simulink model "four_quadrant_chopper"  (R2024b)
settings: Solver=FixedStepAuto  StartTime=0.0  StopTime=1  FixedStep=1e-06  MaxStep=1e-6  RelTol=1e-3
values from neighbouring files (symbols this model uses):
  fsw = 100000    [parameters.m]
  Is = 102    [parameters.m]
  J = Jl + Jr    (= 3.48e-05)    [parameters.m]
  kt = 0.0164    [parameters.m]
  kw = ks*30/pi    (= 5548.14131618)    [parameters.m]
  R = 0.12    [parameters.m]
  Ri = 0.1    [parameters.m]
  Rii = 1000    [parameters.m]
  Rp = 0.02    [parameters.m]
  Rpi = 50    [parameters.m]
  Rv = 0.15    [parameters.m]
  slt = 0.00002848    (= 2.848e-05)    [parameters.m]
  V = 15    [parameters.m]
  vn = 6370    [parameters.m]
libraries: nesl_utility x12, ee_lib x10, fl_lib x8, simulink x2
settings Model: Creator=Samuele  LastModifiedBy=tommymagelli
settings SolverCC: ZeroCrossAlgorithm=Adaptive
settings DebuggingCC: IgnoredZcDiagnostic=none
settings RTWCC: GPUComputeCapability=3.5

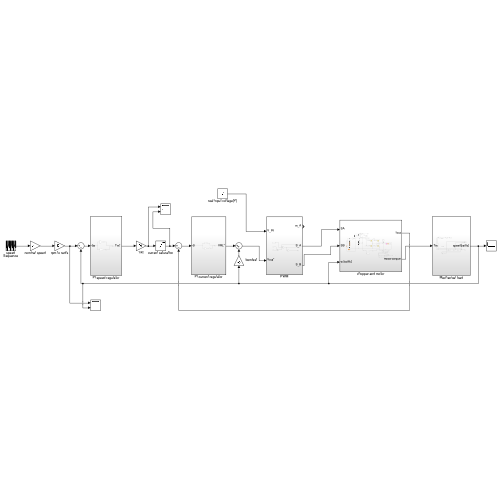
[thumbnail: Simulink's stored preview of the top-level diagram]
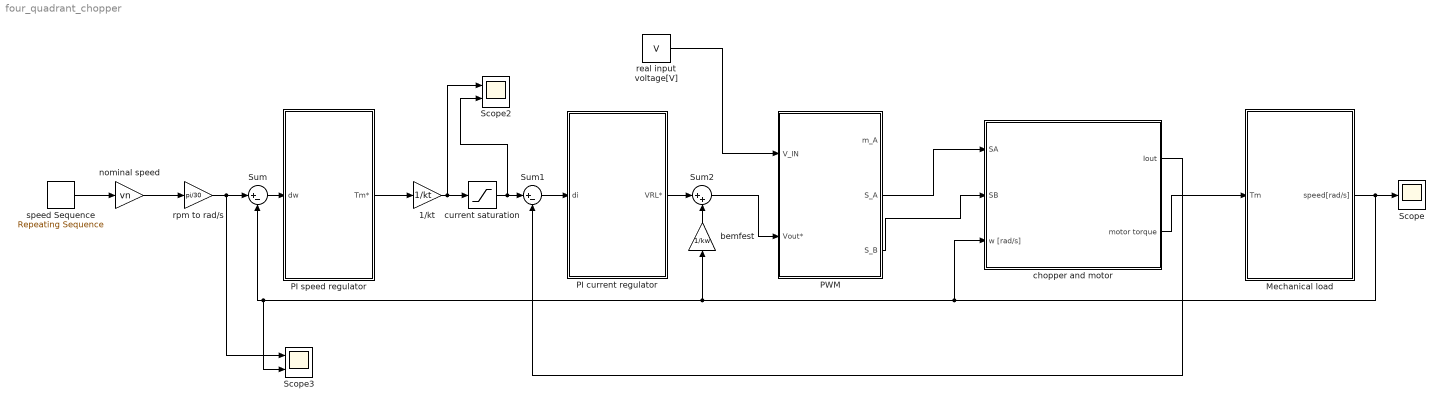
== system four_quadrant_chopper ==
  1/kt : Gain  Gain=1/kt
  Mechanical load : Subsystem
  PI current regulator : Subsystem
  PI speed regulator : Subsystem
  PWM : Subsystem
  Scope : Scope
  Scope2 : Scope  NumInputPorts=2
  Scope3 : Scope  NumInputPorts=2
  Sum : Sum  Inputs=|+-
  Sum1 : Sum  Inputs=|+-
  Sum2 : Sum  Inputs=|++
  bemfest : Gain  Gain=1/kw
  chopper and motor : Subsystem
  current saturation : Saturate  UpperLimit=Is  LowerLimit=-Is
  nominal speed : Gain  Gain=vn
  real input voltage[V] : Constant  Value=V
  rpm to rad/s : Gain  Gain=pi/30
  speed Sequence : simulink/Sources/Repeating Sequence  rep_seq_t=time  rep_seq_y=value
  wires:
  Sum1/1 -> PI current regulator/1(di)
  1/kt/1 -> Scope2/1, current saturation/1
  real input voltage[V]/1 -> PWM/1(V_IN)
  PI speed regulator/1(Tm*) -> 1/kt/1
  Sum2/1 -> PWM/2(Vout*)
  PI current regulator/1(VRL*) -> Sum2/1
  current saturation/1 -> Scope2/2, Sum1/1
  Sum/1 -> PI speed regulator/1(dw)
  rpm to rad/s/1 -> Scope3/1, Sum/1
  speed Sequence/1 -> nominal speed/1
  Mechanical load/1(speed[rad/s]) -> chopper and motor/3(w [rad/s]), Scope3/2, Sum/2, bemfest/1, Scope/1
  nominal speed/1 -> rpm to rad/s/1
  bemfest/1 -> Sum2/2
  chopper and motor/1(Iout) -> Sum1/2
  chopper and motor/2(motor torque) -> Mechanical load/1(Tm)
  PWM/2(S_A) -> chopper and motor/1(SA)
  PWM/3(S_B) -> chopper and motor/2(SB)

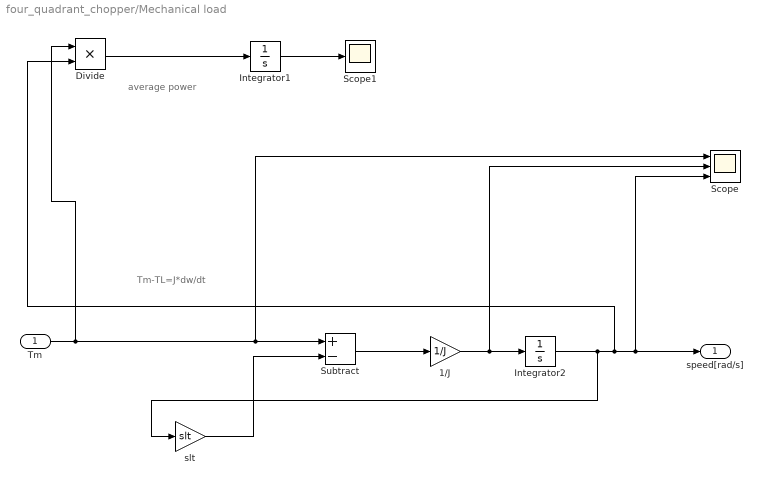
== system four_quadrant_chopper/Mechanical load ==
  note: Tm-TL=J*dw/dt
  note: average power
  Tm : Inport
  1/J : Gain  Gain=1/J
  Divide : Product  Inputs=**
  Integrator1 : Integrator
  Integrator2 : Integrator
  Scope : Scope  NumInputPorts=3
  Scope1 : Scope
  Subtract : Sum  Inputs=+-
  slt : Gain  Gain=slt
  speed[rad/s] : Outport
  wires:
  1/J/1 -> Integrator2/1, Scope/2
  Subtract/1 -> 1/J/1
  Tm/1 -> Divide/1, Scope/1, Subtract/1
  slt/1 -> Subtract/2
  Integrator1/1 -> Scope1/1
  Divide/1 -> Integrator1/1
  Integrator2/1 -> slt/1, Divide/2, Scope/3, speed[rad/s]/1

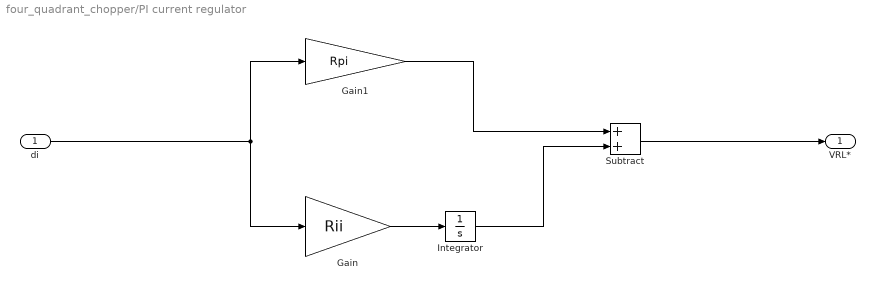
== system four_quadrant_chopper/PI current regulator ==
  di : Inport
  Gain : Gain  Gain=Rii
  Gain1 : Gain  Gain=Rpi
  Integrator : Integrator
  Subtract : Sum
  VRL* : Outport
  wires:
  Integrator/1 -> Subtract/2
  Gain1/1 -> Subtract/1
  Gain/1 -> Integrator/1
  di/1 -> Gain1/1, Gain/1
  Subtract/1 -> VRL*/1

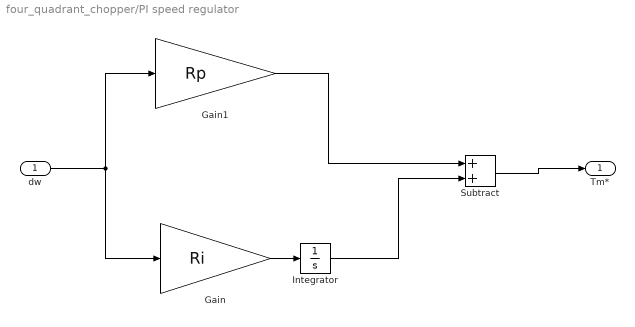
== system four_quadrant_chopper/PI speed regulator ==
  dw : Inport
  Gain : Gain  Gain=Ri
  Gain1 : Gain  Gain=Rp
  Integrator : Integrator
  Subtract : Sum
  Tm* : Outport
  wires:
  Subtract/1 -> Tm*/1
  dw/1 -> Gain1/1, Gain/1
  Gain/1 -> Integrator/1
  Integrator/1 -> Subtract/2
  Gain1/1 -> Subtract/1

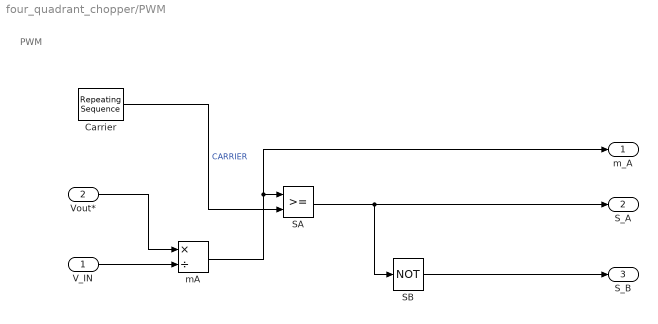
== system four_quadrant_chopper/PWM ==
  note: PWM
  V_IN : Inport
  Vout* : Inport  Port=2
  Carrier : simulink/Sources/Repeating Sequence  rep_seq_t="[0 1/2/fsw  1/fsw]"  rep_seq_y=[-1 1 -1]
  SA : RelationalOperator  OutDataTypeStr=boolean  RndMeth=Simplest  InputSameDT=off
  SB : Logic  Operator=NOT  AllPortsSameDT=off  OutDataTypeStr=boolean
  mA : Product  Inputs=*/
  m_A : Outport
  S_A : Outport  Port=2
  S_B : Outport  Port=3
  wires:
  Carrier/1 -> SA/2  "CARRIER"
  SB/1 -> S_B/1
  SA/1 -> SB/1, S_A/1
  mA/1 -> m_A/1, SA/1
  Vout*/1 -> mA/1
  V_IN/1 -> mA/2

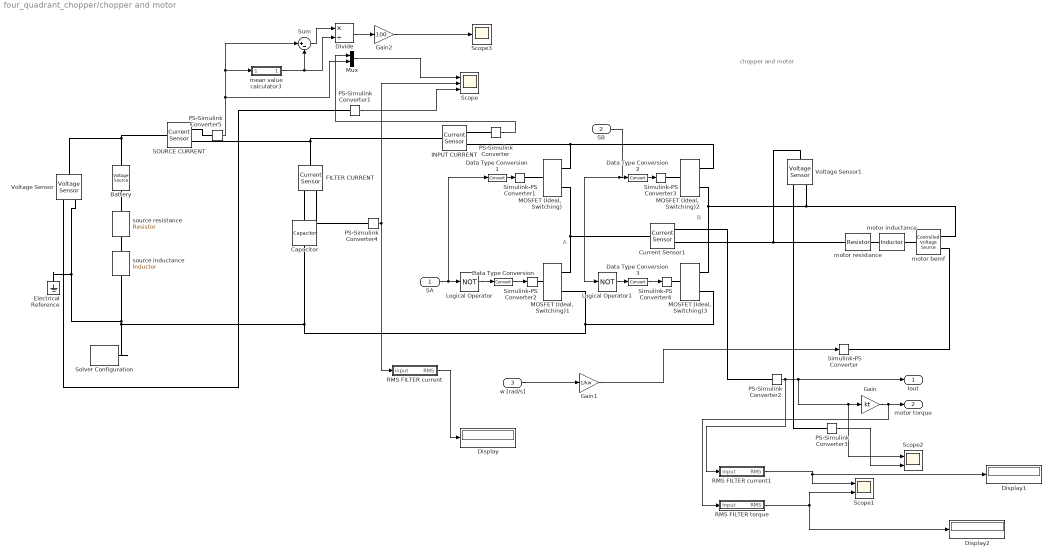
== system four_quadrant_chopper/chopper and motor ==
  note: B
  note: A
  note: chopper and motor
  SA : Inport
  SB : Inport  Port=2
  w [rad/s] : Inport  Port=3
  Battery : ee_lib/Sources/Voltage Source  dc_voltage=V V  ac_voltage=0 V  ac_shift=0 rad  ac_frequency=60 Hz  noise_mode=0  PSD=0 V^2/Hz  sample_time=1e-3 s  repeatability=1  user_seed=0  auto_seed=3499211588  i_specify=off  i_priority=None  i=0 A  i_nominal_specify=off  i_nominal_value=1  i_nominal_unit=A  v_specify=off  v_priority=None  v=0 V  v_nominal_specify=off  v_nominal_value=1  v_nominal_unit=V
  Capacitor : ee_lib/Passive/Capacitor  cap_option=ee.enum.passive.capacitor.capOption.const  c=940e-6 F  Cvec=[1e-05, 1e-06] F  Vvec=[0, 10] V  CV_table_symmetry=1  f_vec=[1, 10] kHz  DFext_vec=[.8, 1.2]  enable_C_tol=0  averaging_period=0 s  C_tol=5  tol_distribution=1  nSigma=4  r=0.21 Ohm  g=0 1/Ohm  enable_operating_limits=0  operating_limit_action=2  max_working_voltage_range=[-25, 25] V  power_rating=1 W  maxTemperature=85 degC  thermalEnable=false  thermalMass=1 J/K  fault_action=simscape.enum.assert.action.none  t_fault=1 s  i_specify=off  i_priority=None  i=0 A  i_nominal_specify=off  i_nominal_value=1  i_nominal_unit=A  v_specify=off  v_priority=None  v=0 V  v_nominal_specify=off  v_nominal_value=1  v_nominal_unit=V  vc_specify=off  vc_priority=High  vc=0 V  vc_nominal_specify=off  vc_nominal_value=1  vc_nominal_unit=V  T_specify=off  T_priority=None  T=298.15 K  T_nominal_specify=off  T_nominal_value=1  T_nominal_unit=K
  Current Sensor1 : fl_lib/Electrical/Electrical Sensors/Current Sensor
  Data Type Conversion{,1..3} (4 alike) : DataTypeConversion  SaturateOnIntegerOverflow=off  RndMeth=Floor
  Display : Display
  Display1 : Display
  Display2 : Display
  Divide : Product  Inputs=*/
  Electrical Reference : fl_lib/Electrical/Electrical Elements/Electrical Reference
  FILTER CURRENT : fl_lib/Electrical/Electrical Sensors/Current Sensor
  Gain : Gain  Gain=kt
  Gain1 : Gain  Gain=1/kw
  Gain2 : Gain  Gain=100
  INPUT CURRENT : fl_lib/Electrical/Electrical Sensors/Current Sensor
  Logical Operator : Logic  Operator=NOT  AllPortsSameDT=off  OutDataTypeStr=boolean
  Logical Operator1 : Logic  Operator=NOT  AllPortsSameDT=off  OutDataTypeStr=boolean
  MOSFET (Ideal, Switching){,1..3} (4 alike) : ee_lib/Semiconductors & Converters/MOSFET (Ideal, Switching)  port_option=ee.enum.controlport.ps  Rds=0.01 Ohm  Goff=1e-6 1/Ohm  Vth=0.5 V  diode_param=1  diode_Vf=0.8 V  diode_Ron=0.001 Ohm  diode_Goff=1e-5 1/Ohm  diode_C=50e-9 F  diode_iRM=-235 A  diode_iF=300 A  diode_idot=-50 A/us  diode_trr_param=1  diode_trr_factor=3  diode_trr=15 us  diode_Qrr=1500 s*uA  ids_specify=off  ids_priority=None  ids=0 A  ids_nominal_specify=off  ids_nominal_value=1  ids_nominal_unit=A  vds_specify=off  vds_priority=None  vds=0 V  vds_nominal_specify=off  vds_nominal_value=1  vds_nominal_unit=V  vgs_specify=off  vgs_priority=None  vgs=0 V  vgs_nominal_specify=off  vgs_nominal_value=1  vgs_nominal_unit=V  thermal_loss_option=ee.enum.converters.thermalLossOption.constantvalues  Von_data=[0, 1.8, 3.2, 6, 10, 16; 0, 2, 5.5, 9.5, 15, 25] V  Tj=[298.15, 448.15] K  Iout_data=[0, 20, 40, 60, 80, 100] A  Eon_data=[0, 55.04, 124.57, 235.53, 362.12; 0, 71.25, 161.25, 304.88, 468.75] * 1e-6 J  Eoff_data=[0, 18, 30, 56.1, 76.5; 0, 22.5, 37.5, 70.13, 95.63] * 1e-6 J  Eon_data_3D=[zeros(2, 5, 3)] J  Eoff_data_3D=[zeros(2, 5, 3)] J  Tj_loss=[298.15, 448.15] K  Iout_data_loss=[0, 10, 20, 30, 40] A  tabulateWithVds=false  Vds_loss=[0, 150, 300] V  Eon_scalar=22.86e-3 J  Eoff_scalar=17.14e-3 J  Voff=300 V  Iout_scalar=600 A  useCurrentFromPreviousCycle=false  useVoltageFromPreviousCycle=false  diodeModelType=ee.enum.converters.diodeModelType.pwl  diodeTableType=ee.enum.diode.tableType.IfMat  diode_ReverseIVType=ee.enum.diode.diodeReverseIV.constant  diode_IfMat=[.07, .12, .19, 1.75, 4.24, 7.32, 11.2; .16, .3, .72, 2.14, 4.02, 6.35, 9.12] A  diode_VfMat=[.9, 1.15, 1.25, 1.5, 1.75, 2.17, 2.6, 2.85; .58, .68, .75, 1.1, 1.38, 1.77, 2.27, 2.7] V  diode_TjVec=[25, 125] degC  diode_VfVec=[.5, .7, .9, 1.3, 1.7, 2.1, 2.5] V  diode_IfVec=[.1, .2, .5, 1, 2, 4, 7, 10] A  diode_IrMat=[1e-06, 2e-06, 5e-06, 1e-05, 2.5e-05, 5e-05, .0001; 2e-06, 5e-06, 1e-05, 4e-05, 8e-05, .0002, .0005] A  diode_VrMat=[10, 100, 200, 250, 300, 325, 350; 10, 70, 160, 220, 270, 300, 320] V  diode_VrVec=[10, 20, 40, 50, 70, 80, 100] V  diode_IrVec=[1e-06, 2e-06, 5e-06, 1e-05, 2e-05, 5e-05, .0001] A  diode_Vr=-600 V  diode_Ls=150 nH  diode_Erec=0.03 J  diode_rec_loss_model=ee.enum.diode.reverseRecoveryModel.fixed  diode_ErecVal=0 J  diode_scaleWithIandV=true  diode_ErecMat=zeros(2, 3) J  diode_TjrecVec=[298.15, 398.15] K  diode_IfrecVec=[.1, 1, 10] A  diode_IrecVal=10 A  diode_VrecVal=10 V  diode_tFilter=1 / 1000 / 100 s  separateThermalPortForDiode=false  thermal_network_parameterization=ee.enum.thermalNetworkTopology.external  Rth=[.03, .2] K/W  Rth_Cauer=[.03, .1, .2] K/W  Rth_Foster=[.03, .2] K/W  thermal_mass_parameterization=ee.enum.thermalNetwork.timeconstant  thermal_mass=[3, 25] J/K  thermal_mass_Cauer=[3, 10, 25] J/K  thermal_mass_Foster=[33, 50] J/K  thermal_time_constant=[.1, 5] s  thermal_time_constant_Cauer=[.1, 1, 5] s  thermal_time_constant_Foster=[1, 10] s  thermal_mass_initial_temperatures=[25, 25] degC  thermal_mass_initial_temperatures_Cauer=[25, 25, 25] degC  junction_thermal_mass=0.1 J/K  Tvec_initial_Foster=[25, 25, 25, 25] degC  RthDiode=[.03, .2] K/W  RthCauerDiode=[.03, .1, .2] K/W  RthFosterDiode=[.03, .2] K/W  thermalMassDiode=[3, 25] J/K  thermalMassCauerDiode=[3, 10, 25] J/K  thermalMassFosterDiode=[33, 50] J/K  thermalTauDiode=[.1, 5] s  thermalTauCauerDiode=[.1, 1, 5] s  thermalTauFosterDiode=[1, 10] s  thermalMassInitTempDiode=[25, 25] degC  thermalMassInitTempCauerDiode=[25, 25, 25] degC  junctionthermalMassDiode=0.1 J/K  TVecInitialFosterDiode=[25, 25, 25, 25] degC  no_thermal_network=0  mosfet_junction_temperature_specify=off  mosfet_junction_temperature_priority=None  mosfet_junction_temperature=25 degC  mosfet_junction_temperature_nominal_specify=off  mosfet_junction_temperature_nominal_value=1  mosfet_junction_temperature_nominal_unit=degC  diode_junction_temperature_specify=off  diode_junction_temperature_priority=None  diode_junction_temperature=25 degC  diode_junction_temperature_nominal_specify=off  diode_junction_temperature_nominal_value=1  diode_junction_temperature_nominal_unit=degC  Qj_specify=off  Qj_priority=None  Qj=0 W  Qj_nominal_specify=off  Qj_nominal_value=1  Qj_nominal_unit=W  accumulatedSwitchingLosses_specify=off  accumulatedSwitchingLosses_priority=None  accumulatedSwitchingLosses=0 J
  Mux : Mux  Inputs=2
  PS-Simulink Converter{,1..5} (6 alike) : nesl_utility/PS-Simulink Converter  PhysicalDomain=network_engine_domain  SubClassName=ps_output  LeftPortType=input  RightPortType=output  PseudoPeriodic=off  Frequencies=[]  VectorFormat=1-D array  Unit=inherit  AffineConversion=off
  RMS FILTER current : Subsystem  mask{t=1/fsw}
      mask prompts: t "Integrating time T [s]"
      mask DialogControl DescTextVar Prompt: Mean value calculator over period T
  RMS FILTER current1 : Subsystem  mask{t=1}
      mask prompts: t "Integrating time T [s]"
      mask DialogControl DescTextVar Prompt: Mean value calculator over period T
  RMS FILTER torque : Subsystem  mask{t=1}
      mask prompts: t "Integrating time T [s]"
      mask DialogControl DescTextVar Prompt: Mean value calculator over period T
  SOURCE CURRENT : fl_lib/Electrical/Electrical Sensors/Current Sensor
  Scope : Scope  NumInputPorts=3
  Scope1 : Scope  NumInputPorts=2
  Scope2 : Scope  NumInputPorts=2
  Scope3 : Scope
  Simulink-PS Converter{,1..4} (5 alike) : nesl_utility/Simulink-PS Converter  PhysicalDomain=network_engine_domain  SubClassName=ps_input  LeftPortType=input  RightPortType=output  PseudoPeriodic=off  Frequencies=[]  NoiseDistribution=none  NoiseParameters=[]  Unit=1  AffineConversion=off  FilteringAndDerivatives=provide  SimscapeFilterOrder=1  InputFilterTimeConstant=0.001  UdotUserProvided=0
  Solver Configuration : nesl_utility/Solver Configuration  PhysicalDomain=network_engine_domain  SubClassName=solver  LeftPortType=input  RightPortType=generic  Tones=[]  Harmonics=[]  SimulateNoise=off  Profile=off  UseLocalSampling=off  EnableSwitchedLinearOptims=on  FrequencyDomain=off  UseCCode=off  RelTol=0.001  AbsTol=1e-06  MinStep=1e-09  ToWorkspace=off  RevertToSquareIcSolve=off  NumHomotopyIterations=100  PhasorMode=off  PhasorModeNumHarmonics=1  ConsistencySolver=NEWTON_FTOL  IndexReductionMethod=DerivativeReplacement  DoDC=off  ResidualTolerance=1e-09  ConsistencyTolSource=GLOBAL  ConsistencyAbsTol=0.001  ConsistencyRelTol=0.001  ConsistencyTolFactor=0.001  UseLocalSolver=off  LocalSolverChoice=NE_BACKWARD_EULER_ADVANCER  ResolveIndetEquations=on  FunctionEvalNumThread=1  LocalSolverSampleTime=0.001  DoFixedCost=off  MaxNonlinIter=3  MaxModeIter=2  ComputeImpulses=off  ImpulseIterations=2  LinearAlgebra=auto  LinearAlgebraNumThread=0  EquationFormulation=NE_TIME_EF  DelaysMemoryBudget=1024  AutomaticFiltering=on  FilteringTimeConstant=0.001  PartitionStorageMethod=AS_NEEDED  PartitionMemoryBudget=1024  PartitionMethod=ROBUST  MultibodyUseLocalSolver=off  MultibodyLocalSolverChoice=ODE1  MultibodyLocalSolverSampleTime=0.001
  Sum : Sum  Inputs=|+-
  Voltage Sensor : fl_lib/Electrical/Electrical Sensors/Voltage Sensor
  Voltage Sensor1 : fl_lib/Electrical/Electrical Sensors/Voltage Sensor
  mean value calculator3 : Subsystem  mask{t=1/500000}
      mask prompts: t "Integrating time T [s]"
      mask DialogControl DescTextVar Prompt: Mean value calculator over period T
  motor inductance : ee_lib/Passive/Inductor  l=L H  enable_L_tol=0  L_tol=20  tol_distribution=1  nSigma=4  r=0 Ohm  g=1e-9 1/Ohm  enable_operating_limits=0  operating_limit_action=2  max_working_current=1 A  power_rating=1 W  fault_action=simscape.enum.assert.action.none  t_fault=1 s  i_L_specify=off  i_L_priority=High  i_L=0 A  i_L_nominal_specify=off  i_L_nominal_value=1  i_L_nominal_unit=A
  "motor resistance " : ee_lib/Passive/Resistor  R=R Ohm  enable_R_tol=0  R_tol=5  tol_distribution=1  nSigma=4  enable_operating_limits=0  operating_limit_action=2  power_rating=1 W  max_working_voltage=100 V  noise_mode=0  Tdevice=25 degC  sample_time=1e-3 s  repeatability=1  user_seed=0  auto_seed=3890346746  fault_action=simscape.enum.assert.action.none  t_fault=1 s  power_derating_T1=70 degC  power_derating_T2=155 degC  operating_temperature_range_vec=[-50, 150] degC  alpha=3.93e-3 1/K  Tmeas=25 degC  thermal_mass=100 J/K  temperature_specify=off  temperature_priority=High  temperature=298.15 K  temperature_nominal_specify=off  temperature_nominal_value=1  temperature_nominal_unit=K
  motor bemf : fl_lib/Electrical/Electrical Sources/Controlled Voltage Source
  source inductance : ee_lib/Passive/Inductor  l=Lv H  enable_L_tol=0  L_tol=20  tol_distribution=1  nSigma=4  r=0 Ohm  g=1e-9 1/Ohm  enable_operating_limits=0  operating_limit_action=2  max_working_current=1 A  power_rating=1 W  fault_action=simscape.enum.assert.action.none  t_fault=1 s  i_L_specify=off  i_L_priority=High  i_L=0 A  i_L_nominal_specify=off  i_L_nominal_value=1  i_L_nominal_unit=A
  source resistance : ee_lib/Passive/Resistor  R=Rv Ohm  enable_R_tol=0  R_tol=5  tol_distribution=1  nSigma=4  enable_operating_limits=0  operating_limit_action=2  power_rating=1 W  max_working_voltage=100 V  noise_mode=0  Tdevice=25 degC  sample_time=1e-3 s  repeatability=1  user_seed=0  auto_seed=545404223  fault_action=simscape.enum.assert.action.none  t_fault=1 s  power_derating_T1=70 degC  power_derating_T2=155 degC  operating_temperature_range_vec=[-50, 150] degC  alpha=3.93e-3 1/K  Tmeas=25 degC  thermal_mass=100 J/K  temperature_specify=off  temperature_priority=High  temperature=298.15 K  temperature_nominal_specify=off  temperature_nominal_value=1  temperature_nominal_unit=K
  Iout : Outport
  motor torque : Outport  Port=2
  wires:
  Gain1/1 -> Simulink-PS Converter/1
  PS-Simulink Converter1/1 -> Scope/3
  RMS FILTER current/1(RMS) -> Display/1
  PS-Simulink Converter4/1 -> RMS FILTER current/1(input), Scope/2
  Data Type Conversion3/1 -> Simulink-PS Converter4/1
  Mux/1 -> Scope/1
  PS-Simulink Converter/1 -> Mux/1
  w [rad/s]/1 -> Gain1/1
  Data Type Conversion2/1 -> Simulink-PS Converter3/1
  Logical Operator1/1 -> Data Type Conversion3/1
  PS-Simulink Converter3/1 -> Scope2/2
  Gain/1 -> RMS FILTER torque/1(input), motor torque/1
  Logical Operator/1 -> Data Type Conversion/1
  SA/1 -> Data Type Conversion1/1, Logical Operator/1
  Data Type Conversion/1 -> Simulink-PS Converter2/1
  Data Type Conversion1/1 -> Simulink-PS Converter1/1
  SB/1 -> Logical Operator1/1, Data Type Conversion2/1
  PS-Simulink Converter2/1 -> RMS FILTER current1/1(input), Scope2/1, Gain/1, Iout/1
  RMS FILTER torque/1(RMS) -> Scope1/2, Display2/1
  RMS FILTER current1/1(RMS) -> Display1/1, Scope1/1
  PS-Simulink Converter5/1 -> Mux/2, mean value calculator3/1(input), Sum/1
  Sum/1 -> Divide/1
  Divide/1 -> Gain2/1
  Gain2/1 -> Scope3/1
  mean value calculator3/1(mean) -> Divide/2, Sum/2
  connections:
  Current Sensor1/LConn1 -- "MOSFET (Ideal, Switching)"/RConn2 -- "MOSFET (Ideal, Switching)1"/RConn1
  "MOSFET (Ideal, Switching)3"/RConn2 -- Capacitor/RConn1 -- source inductance/RConn1 -- Electrical Reference/LConn1 -- Voltage Sensor/RConn2 -- Solver Configuration/RConn1 -- "MOSFET (Ideal, Switching)1"/RConn2
  INPUT CURRENT/LConn1 -- FILTER CURRENT/LConn1 -- SOURCE CURRENT/RConn2
  Voltage Sensor1/LConn1 -- Current Sensor1/RConn2 -- "motor resistance "/LConn1
  Voltage Sensor1/RConn2 -- "MOSFET (Ideal, Switching)3"/RConn1 -- "MOSFET (Ideal, Switching)2"/RConn2 -- motor bemf/RConn2
  "MOSFET (Ideal, Switching)"/RConn1 -- INPUT CURRENT/RConn2 -- "MOSFET (Ideal, Switching)2"/RConn1
  SOURCE CURRENT/LConn1 -- Voltage Sensor/LConn1 -- Battery/LConn1
  FILTER CURRENT/RConn2 -- Capacitor/LConn1
  source inductance/LConn1 -- source resistance/RConn1
  SOURCE CURRENT/RConn1 -- PS-Simulink Converter5/LConn1
  Simulink-PS Converter4/RConn1 -- "MOSFET (Ideal, Switching)3"/LConn1
  Simulink-PS Converter1/RConn1 -- "MOSFET (Ideal, Switching)"/LConn1
  Voltage Sensor1/RConn1 -- PS-Simulink Converter3/LConn1
  FILTER CURRENT/RConn1 -- PS-Simulink Converter4/LConn1
  Current Sensor1/RConn1 -- PS-Simulink Converter2/LConn1
  Voltage Sensor/RConn1 -- PS-Simulink Converter1/LConn1
  Simulink-PS Converter2/RConn1 -- "MOSFET (Ideal, Switching)1"/LConn1
  motor inductance/RConn1 -- motor bemf/LConn1
  INPUT CURRENT/RConn1 -- PS-Simulink Converter/LConn1
  "motor resistance "/RConn1 -- motor inductance/LConn1
  source resistance/LConn1 -- Battery/RConn1
  Simulink-PS Converter3/RConn1 -- "MOSFET (Ideal, Switching)2"/LConn1
  Simulink-PS Converter/RConn1 -- motor bemf/RConn1

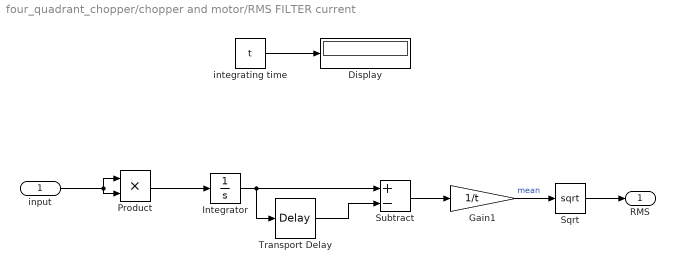
== system four_quadrant_chopper/chopper and motor/RMS FILTER current ==
  input : Inport
  Display : Display
  Gain1 : Gain  Gain=1/t
  Integrator : Integrator
  Product : Product
  Sqrt : Sqrt
  Subtract : Sum  Inputs=+-
  Transport Delay : TransportDelay  DelayTime=t
  integrating time : Constant  Value=t
  RMS : Outport
  wires:
  integrating time/1 -> Display/1
  Transport Delay/1 -> Subtract/2
  Integrator/1 -> Transport Delay/1, Subtract/1
  Subtract/1 -> Gain1/1
  input/1 -> Product/1, Product/2
  Product/1 -> Integrator/1
  Sqrt/1 -> RMS/1
  Gain1/1 -> Sqrt/1  "mean"

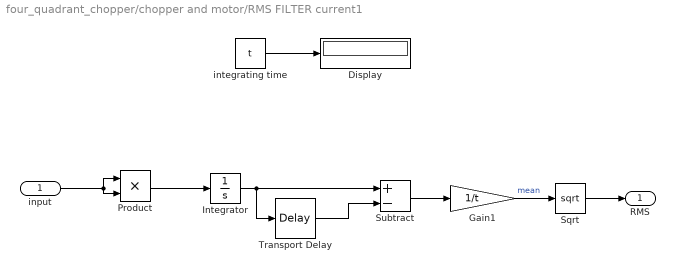
== system four_quadrant_chopper/chopper and motor/RMS FILTER current1 ==
  input : Inport
  Display : Display
  Gain1 : Gain  Gain=1/t
  Integrator : Integrator
  Product : Product
  Sqrt : Sqrt
  Subtract : Sum  Inputs=+-
  Transport Delay : TransportDelay  DelayTime=t
  integrating time : Constant  Value=t
  RMS : Outport
  wires:
  integrating time/1 -> Display/1
  Transport Delay/1 -> Subtract/2
  Integrator/1 -> Transport Delay/1, Subtract/1
  Subtract/1 -> Gain1/1
  input/1 -> Product/1, Product/2
  Product/1 -> Integrator/1
  Sqrt/1 -> RMS/1
  Gain1/1 -> Sqrt/1  "mean"

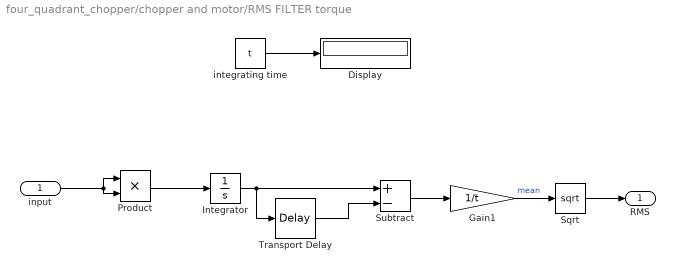
== system four_quadrant_chopper/chopper and motor/RMS FILTER torque ==
  input : Inport
  Display : Display
  Gain1 : Gain  Gain=1/t
  Integrator : Integrator
  Product : Product
  Sqrt : Sqrt
  Subtract : Sum  Inputs=+-
  Transport Delay : TransportDelay  DelayTime=t
  integrating time : Constant  Value=t
  RMS : Outport
  wires:
  integrating time/1 -> Display/1
  Transport Delay/1 -> Subtract/2
  Integrator/1 -> Transport Delay/1, Subtract/1
  Subtract/1 -> Gain1/1
  input/1 -> Product/1, Product/2
  Product/1 -> Integrator/1
  Sqrt/1 -> RMS/1
  Gain1/1 -> Sqrt/1  "mean"

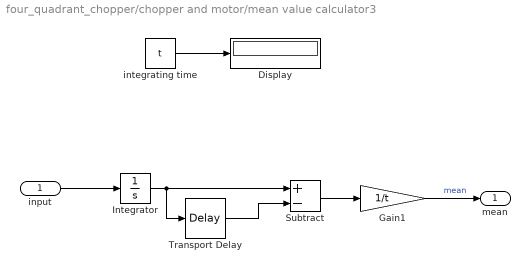
== system four_quadrant_chopper/chopper and motor/mean value calculator3 ==
  input : Inport
  Display : Display
  Gain1 : Gain  Gain=1/t
  Integrator : Integrator
  Subtract : Sum  Inputs=+-
  Transport Delay : TransportDelay  DelayTime=t
  integrating time : Constant  Value=t
  mean : Outport
  wires:
  integrating time/1 -> Display/1
  Transport Delay/1 -> Subtract/2
  Gain1/1 -> mean/1  "mean"
  Integrator/1 -> Transport Delay/1, Subtract/1
  input/1 -> Integrator/1
  Subtract/1 -> Gain1/1
